simulink model "gtm_design"  (R2021b)
settings: Solver=VariableStepAuto  StartTime=0.0  StopTime=10.0  MinStep=0.00999  RelTol=1e-3
StopFcn:
  | MWSout=grabmws(bdroot);
  | MWSout.lastrun=datestr(now);
values from neighbouring files (symbols this model uses):
  knots2fps = 1.68781    [setup.m]
  s = tf('s')    [setup.m]
undefined symbols (not defined in the file or in its folder): Aero, aftfuel, aftfuel_pos, AILL, AILLC, AILR, AILRC, alpha_deg, alt0, altitude_ft, Ax_g, Ay_g, Az_g, b, beta_deg, bias, BRAKEC, Cbar, cg_pos0, cg_shift_gear, ControlMode, DamageCase, DamageModels, DamageOnsetTime, deltc, Earth, ELLIB, ELLIBC, ELLOB, ELLOBC, ELRIB, ELRIBC, ELROB, ELROBC, engl_ang, engl_pos, engr_ang, engr_pos, etas0, etas1, etasc_feedthrough, FLAPLC, FLAPLIB, FLAPLOB, FLAPRC, FLAPRIB, FLAPROB, FlightMode, FuelUsed_Init, fwdfuel, fwdfuel_pos, GEAR, GEARC, Inertia0, Inertia_shift_gear, Ixx_model, Iyy_model, Izz_model, KTAS, LandingGear ... (+66)
libraries: simulink_extras x98, LPVBlockLibrary x54, simulink_need_slupdate x30, aerolibconvert2 x27, simulink x7, aerolibtransform2 x6, uavalgslib x4, UserContent_lib x2, robotcorelib x1, uavutilslib x1
(part 3 of 9)

== system gtm_design/GTM_T2/Actuators/Acutator Dynamics ==
  In : Inport
  Brake : Saturate  UpperLimit=100  LowerLimit=0
  Bus Selector2 : BusSelector  OutputSignals=ELLOBC,ELLIBC,ELROBC,ELRIBC,AILLC,AILRC,RUDUPC,RUDLOC,SPLLIBC,SPLLOBC,SPLRIBC,SPLROBC,FLAPLC,MORPHLC,FLAPRC,MORPHRC,GEARC,BRAKEC,THROTLC,THROTRC,STEERC
  ElevatorLIBServo : Subsystem  mask(Rate and Position Limited Servo){freq=5, RL=300, POS_hi=20, POS_lo=-30, Bias=bias.elevator}
      mask prompts: freq "Bandwidth, Hz"; RL "Rate Limit:"; POS_hi "Position Limit High:"; POS_lo "Position Limit Low:"; Bias "Bias Value:"
      mask help:
      | First order transfer function: w/(s+w), with rate and position limits
      | and output bias level.
      mask Display:
      | text(.48,.55,sprintf('%3.1f Hz\nBW',freq),'horizontalAlignment','center');
      | 
      | text(0.18,0.45,sprintf('|d/dt|\n<%0.1f',RL),'horizontalAlignment','center');
      | 
      | text(0.88,0.85,num2str(POS_hi),'horizontalAlignment', 'center');
      | text(0.88,0.2,num2str(POS_lo),'horizontalAlignment', 'center');
      | text(0.73,0.5,'P\nL');
      | 
      | 
      | plot([0.83 0.87 0.93 0.97],[0.4 0.4 0.6 0.6]);
      | plot([0.81 0.99],[0.5 0.5]);
      | plot([0.9 0.9],[0.3 0.7]);
      | plot([0.81 0.99 0.99 0.81 0.81],[0.3 0.3 0.7 0.7 0.3]);
  ElevatorLOBServo : Subsystem  mask(Rate and Position Limited Servo){freq=5, RL=300, POS_hi=20, POS_lo=-30, Bias=bias.elevator}
      mask prompts: freq "Bandwidth, Hz"; RL "Rate Limit:"; POS_hi "Position Limit High:"; POS_lo "Position Limit Low:"; Bias "Bias Value:"
      mask help:
      | First order transfer function: w/(s+w), with rate and position limits
      | and output bias level.
      mask Display:
      | text(.48,.55,sprintf('%3.1f Hz\nBW',freq),'horizontalAlignment','center');
      | 
      | text(0.18,0.45,sprintf('|d/dt|\n<%0.1f',RL),'horizontalAlignment','center');
      | 
      | text(0.88,0.85,num2str(POS_hi),'horizontalAlignment', 'center');
      | text(0.88,0.2,num2str(POS_lo),'horizontalAlignment', 'center');
      | text(0.73,0.5,'P\nL');
      | 
      | 
      | plot([0.83 0.87 0.93 0.97],[0.4 0.4 0.6 0.6]);
      | plot([0.81 0.99],[0.5 0.5]);
      | plot([0.9 0.9],[0.3 0.7]);
      | plot([0.81 0.99 0.99 0.81 0.81],[0.3 0.3 0.7 0.7 0.3]);
  ElevatorRIBServo : Subsystem  mask(Rate and Position Limited Servo){freq=5, RL=300, POS_hi=20, POS_lo=-30, Bias=bias.elevator}
      mask prompts: freq "Bandwidth, Hz"; RL "Rate Limit:"; POS_hi "Position Limit High:"; POS_lo "Position Limit Low:"; Bias "Bias Value:"
      mask help:
      | First order transfer function: w/(s+w), with rate and position limits
      | and output bias level.
      mask Display:
      | text(.48,.55,sprintf('%3.1f Hz\nBW',freq),'horizontalAlignment','center');
      | 
      | text(0.18,0.45,sprintf('|d/dt|\n<%0.1f',RL),'horizontalAlignment','center');
      | 
      | text(0.88,0.85,num2str(POS_hi),'horizontalAlignment', 'center');
      | text(0.88,0.2,num2str(POS_lo),'horizontalAlignment', 'center');
      | text(0.73,0.5,'P\nL');
      | 
      | 
      | plot([0.83 0.87 0.93 0.97],[0.4 0.4 0.6 0.6]);
      | plot([0.81 0.99],[0.5 0.5]);
      | plot([0.9 0.9],[0.3 0.7]);
      | plot([0.81 0.99 0.99 0.81 0.81],[0.3 0.3 0.7 0.7 0.3]);
  ElevatorROBServo : Subsystem  mask(Rate and Position Limited Servo){freq=5, RL=300, POS_hi=20, POS_lo=-30, Bias=bias.elevator}
      mask prompts: freq "Bandwidth, Hz"; RL "Rate Limit:"; POS_hi "Position Limit High:"; POS_lo "Position Limit Low:"; Bias "Bias Value:"
      mask help:
      | First order transfer function: w/(s+w), with rate and position limits
      | and output bias level.
      mask Display:
      | text(.48,.55,sprintf('%3.1f Hz\nBW',freq),'horizontalAlignment','center');
      | 
      | text(0.18,0.45,sprintf('|d/dt|\n<%0.1f',RL),'horizontalAlignment','center');
      | 
      | text(0.88,0.85,num2str(POS_hi),'horizontalAlignment', 'center');
      | text(0.88,0.2,num2str(POS_lo),'horizontalAlignment', 'center');
      | text(0.73,0.5,'P\nL');
      | 
      | 
      | plot([0.83 0.87 0.93 0.97],[0.4 0.4 0.6 0.6]);
      | plot([0.81 0.99],[0.5 0.5]);
      | plot([0.9 0.9],[0.3 0.7]);
      | plot([0.81 0.99 0.99 0.81 0.81],[0.3 0.3 0.7 0.7 0.3]);
  FlapLServo : Subsystem  mask(Rate and Position Limited Servo){freq=5, RL=300, POS_hi=30, POS_lo=0, Bias=bias.morphing}
      mask prompts: freq "Bandwidth, Hz"; RL "Rate Limit:"; POS_hi "Position Limit High:"; POS_lo "Position Limit Low:"; Bias "Bias Value:"
      mask help:
      | First order transfer function: w/(s+w), with rate and position limits
      | and output bias level.
      mask Display:
      | text(.48,.55,sprintf('%3.1f Hz\nBW',freq),'horizontalAlignment','center');
      | 
      | text(0.18,0.45,sprintf('|d/dt|\n<%0.1f',RL),'horizontalAlignment','center');
      | 
      | text(0.88,0.85,num2str(POS_hi),'horizontalAlignment', 'center');
      | text(0.88,0.2,num2str(POS_lo),'horizontalAlignment', 'center');
      | text(0.73,0.5,'P\nL');
      | 
      | 
      | plot([0.83 0.87 0.93 0.97],[0.4 0.4 0.6 0.6]);
      | plot([0.81 0.99],[0.5 0.5]);
      | plot([0.9 0.9],[0.3 0.7]);
      | plot([0.81 0.99 0.99 0.81 0.81],[0.3 0.3 0.7 0.7 0.3]);
  FlapRServo : Subsystem  mask(Rate and Position Limited Servo){freq=5, RL=300, POS_hi=30, POS_lo=0, Bias=bias.morphing}
      mask prompts: freq "Bandwidth, Hz"; RL "Rate Limit:"; POS_hi "Position Limit High:"; POS_lo "Position Limit Low:"; Bias "Bias Value:"
      mask help:
      | First order transfer function: w/(s+w), with rate and position limits
      | and output bias level.
      mask Display:
      | text(.48,.55,sprintf('%3.1f Hz\nBW',freq),'horizontalAlignment','center');
      | 
      | text(0.18,0.45,sprintf('|d/dt|\n<%0.1f',RL),'horizontalAlignment','center');
      | 
      | text(0.88,0.85,num2str(POS_hi),'horizontalAlignment', 'center');
      | text(0.88,0.2,num2str(POS_lo),'horizontalAlignment', 'center');
      | text(0.73,0.5,'P\nL');
      | 
      | 
      | plot([0.83 0.87 0.93 0.97],[0.4 0.4 0.6 0.6]);
      | plot([0.81 0.99],[0.5 0.5]);
      | plot([0.9 0.9],[0.3 0.7]);
      | plot([0.81 0.99 0.99 0.81 0.81],[0.3 0.3 0.7 0.7 0.3]);
  Gear : Saturate  UpperLimit=1  LowerLimit=0
  L Throttle : Saturate  UpperLimit=100  LowerLimit=0
  LeftAileronServo : Subsystem  mask(Rate and Position Limited Servo){freq=5, RL=300, POS_hi=20.0, POS_lo=-20, Bias=-1*bias.aileron}
      mask prompts: freq "Bandwidth, Hz"; RL "Rate Limit:"; POS_hi "Position Limit High:"; POS_lo "Position Limit Low:"; Bias "Bias Value:"
      mask help:
      | First order transfer function: w/(s+w), with rate and position limits
      | and output bias level.
      mask Display:
      | text(.48,.55,sprintf('%3.1f Hz\nBW',freq),'horizontalAlignment','center');
      | 
      | text(0.18,0.45,sprintf('|d/dt|\n<%0.1f',RL),'horizontalAlignment','center');
      | 
      | text(0.88,0.85,num2str(POS_hi),'horizontalAlignment', 'center');
      | text(0.88,0.2,num2str(POS_lo),'horizontalAlignment', 'center');
      | text(0.73,0.5,'P\nL');
      | 
      | 
      | plot([0.83 0.87 0.93 0.97],[0.4 0.4 0.6 0.6]);
      | plot([0.81 0.99],[0.5 0.5]);
      | plot([0.9 0.9],[0.3 0.7]);
      | plot([0.81 0.99 0.99 0.81 0.81],[0.3 0.3 0.7 0.7 0.3]);
  LeftIBSpoilerServo : Subsystem  mask(Rate and Position Limited Servo){freq=5, RL=300, POS_hi=15, POS_lo=0, Bias=bias.morphing}
      mask prompts: freq "Bandwidth, Hz"; RL "Rate Limit:"; POS_hi "Position Limit High:"; POS_lo "Position Limit Low:"; Bias "Bias Value:"
      mask help:
      | First order transfer function: w/(s+w), with rate and position limits
      | and output bias level.
      mask Display:
      | text(.48,.55,sprintf('%3.1f Hz\nBW',freq),'horizontalAlignment','center');
      | 
      | text(0.18,0.45,sprintf('|d/dt|\n<%0.1f',RL),'horizontalAlignment','center');
      | 
      | text(0.88,0.85,num2str(POS_hi),'horizontalAlignment', 'center');
      | text(0.88,0.2,num2str(POS_lo),'horizontalAlignment', 'center');
      | text(0.73,0.5,'P\nL');
      | 
      | 
      | plot([0.83 0.87 0.93 0.97],[0.4 0.4 0.6 0.6]);
      | plot([0.81 0.99],[0.5 0.5]);
      | plot([0.9 0.9],[0.3 0.7]);
      | plot([0.81 0.99 0.99 0.81 0.81],[0.3 0.3 0.7 0.7 0.3]);
  LeftOBSpoilerServo : Subsystem  mask(Rate and Position Limited Servo){freq=5, RL=300, POS_hi=45, POS_lo=0, Bias=bias.speedbrake}
      mask prompts: freq "Bandwidth, Hz"; RL "Rate Limit:"; POS_hi "Position Limit High:"; POS_lo "Position Limit Low:"; Bias "Bias Value:"
      mask help:
      | First order transfer function: w/(s+w), with rate and position limits
      | and output bias level.
      mask Display:
      | text(.48,.55,sprintf('%3.1f Hz\nBW',freq),'horizontalAlignment','center');
      | 
      | text(0.18,0.45,sprintf('|d/dt|\n<%0.1f',RL),'horizontalAlignment','center');
      | 
      | text(0.88,0.85,num2str(POS_hi),'horizontalAlignment', 'center');
      | text(0.88,0.2,num2str(POS_lo),'horizontalAlignment', 'center');
      | text(0.73,0.5,'P\nL');
      | 
      | 
      | plot([0.83 0.87 0.93 0.97],[0.4 0.4 0.6 0.6]);
      | plot([0.81 0.99],[0.5 0.5]);
      | plot([0.9 0.9],[0.3 0.7]);
      | plot([0.81 0.99 0.99 0.81 0.81],[0.3 0.3 0.7 0.7 0.3]);
  LeftSpanServo : Subsystem  mask(Rate and Position Limited Servo){freq=5, RL=25, POS_hi=0, POS_lo=-25, Bias=bias.morphing}
      mask prompts: freq "Bandwidth, Hz"; RL "Rate Limit:"; POS_hi "Position Limit High:"; POS_lo "Position Limit Low:"; Bias "Bias Value:"
      mask help:
      | First order transfer function: w/(s+w), with rate and position limits
      | and output bias level.
      mask Display:
      | text(.48,.55,sprintf('%3.1f Hz\nBW',freq),'horizontalAlignment','center');
      | 
      | text(0.18,0.45,sprintf('|d/dt|\n<%0.1f',RL),'horizontalAlignment','center');
      | 
      | text(0.88,0.85,num2str(POS_hi),'horizontalAlignment', 'center');
      | text(0.88,0.2,num2str(POS_lo),'horizontalAlignment', 'center');
      | text(0.73,0.5,'P\nL');
      | 
      | 
      | plot([0.83 0.87 0.93 0.97],[0.4 0.4 0.6 0.6]);
      | plot([0.81 0.99],[0.5 0.5]);
      | plot([0.9 0.9],[0.3 0.7]);
      | plot([0.81 0.99 0.99 0.81 0.81],[0.3 0.3 0.7 0.7 0.3]);
  Mux : Mux  Inputs=21
  R Throttle : Saturate  UpperLimit=100  LowerLimit=0
  RightAileronServo : Subsystem  mask(Rate and Position Limited Servo){freq=5, RL=300, POS_hi=20.0, POS_lo=-20, Bias=bias.aileron}
      mask prompts: freq "Bandwidth, Hz"; RL "Rate Limit:"; POS_hi "Position Limit High:"; POS_lo "Position Limit Low:"; Bias "Bias Value:"
      mask help:
      | First order transfer function: w/(s+w), with rate and position limits
      | and output bias level.
      mask Display:
      | text(.48,.55,sprintf('%3.1f Hz\nBW',freq),'horizontalAlignment','center');
      | 
      | text(0.18,0.45,sprintf('|d/dt|\n<%0.1f',RL),'horizontalAlignment','center');
      | 
      | text(0.88,0.85,num2str(POS_hi),'horizontalAlignment', 'center');
      | text(0.88,0.2,num2str(POS_lo),'horizontalAlignment', 'center');
      | text(0.73,0.5,'P\nL');
      | 
      | 
      | plot([0.83 0.87 0.93 0.97],[0.4 0.4 0.6 0.6]);
      | plot([0.81 0.99],[0.5 0.5]);
      | plot([0.9 0.9],[0.3 0.7]);
      | plot([0.81 0.99 0.99 0.81 0.81],[0.3 0.3 0.7 0.7 0.3]);
  RightIBSpoilerServo : Subsystem  mask(Rate and Position Limited Servo){freq=5, RL=300, POS_hi=15, POS_lo=0, Bias=bias.morphing}
      mask prompts: freq "Bandwidth, Hz"; RL "Rate Limit:"; POS_hi "Position Limit High:"; POS_lo "Position Limit Low:"; Bias "Bias Value:"
      mask help:
      | First order transfer function: w/(s+w), with rate and position limits
      | and output bias level.
      mask Display:
      | text(.48,.55,sprintf('%3.1f Hz\nBW',freq),'horizontalAlignment','center');
      | 
      | text(0.18,0.45,sprintf('|d/dt|\n<%0.1f',RL),'horizontalAlignment','center');
      | 
      | text(0.88,0.85,num2str(POS_hi),'horizontalAlignment', 'center');
      | text(0.88,0.2,num2str(POS_lo),'horizontalAlignment', 'center');
      | text(0.73,0.5,'P\nL');
      | 
      | 
      | plot([0.83 0.87 0.93 0.97],[0.4 0.4 0.6 0.6]);
      | plot([0.81 0.99],[0.5 0.5]);
      | plot([0.9 0.9],[0.3 0.7]);
      | plot([0.81 0.99 0.99 0.81 0.81],[0.3 0.3 0.7 0.7 0.3]);
  RightOBSpoilerServo : Subsystem  mask(Rate and Position Limited Servo){freq=5, RL=300, POS_hi=45, POS_lo=0, Bias=bias.speedbrake}
      mask prompts: freq "Bandwidth, Hz"; RL "Rate Limit:"; POS_hi "Position Limit High:"; POS_lo "Position Limit Low:"; Bias "Bias Value:"
      mask help:
      | First order transfer function: w/(s+w), with rate and position limits
      | and output bias level.
      mask Display:
      | text(.48,.55,sprintf('%3.1f Hz\nBW',freq),'horizontalAlignment','center');
      | 
      | text(0.18,0.45,sprintf('|d/dt|\n<%0.1f',RL),'horizontalAlignment','center');
      | 
      | text(0.88,0.85,num2str(POS_hi),'horizontalAlignment', 'center');
      | text(0.88,0.2,num2str(POS_lo),'horizontalAlignment', 'center');
      | text(0.73,0.5,'P\nL');
      | 
      | 
      | plot([0.83 0.87 0.93 0.97],[0.4 0.4 0.6 0.6]);
      | plot([0.81 0.99],[0.5 0.5]);
      | plot([0.9 0.9],[0.3 0.7]);
      | plot([0.81 0.99 0.99 0.81 0.81],[0.3 0.3 0.7 0.7 0.3]);
  RightSpanServo : Subsystem  mask(Rate and Position Limited Servo){freq=5, RL=25, POS_hi=0, POS_lo=-25, Bias=bias.morphing}
      mask prompts: freq "Bandwidth, Hz"; RL "Rate Limit:"; POS_hi "Position Limit High:"; POS_lo "Position Limit Low:"; Bias "Bias Value:"
      mask help:
      | First order transfer function: w/(s+w), with rate and position limits
      | and output bias level.
      mask Display:
      | text(.48,.55,sprintf('%3.1f Hz\nBW',freq),'horizontalAlignment','center');
      | 
      | text(0.18,0.45,sprintf('|d/dt|\n<%0.1f',RL),'horizontalAlignment','center');
      | 
      | text(0.88,0.85,num2str(POS_hi),'horizontalAlignment', 'center');
      | text(0.88,0.2,num2str(POS_lo),'horizontalAlignment', 'center');
      | text(0.73,0.5,'P\nL');
      | 
      | 
      | plot([0.83 0.87 0.93 0.97],[0.4 0.4 0.6 0.6]);
      | plot([0.81 0.99],[0.5 0.5]);
      | plot([0.9 0.9],[0.3 0.7]);
      | plot([0.81 0.99 0.99 0.81 0.81],[0.3 0.3 0.7 0.7 0.3]);
  RudderLServo : Subsystem  mask(Rate and Position Limited Servo){freq=5, RL=300, POS_hi=30, POS_lo=-30.0, Bias=bias.rudder}
      mask prompts: freq "Bandwidth, Hz"; RL "Rate Limit:"; POS_hi "Position Limit High:"; POS_lo "Position Limit Low:"; Bias "Bias Value:"
      mask help:
      | First order transfer function: w/(s+w), with rate and position limits
      | and output bias level.
      mask Display:
      | text(.48,.55,sprintf('%3.1f Hz\nBW',freq),'horizontalAlignment','center');
      | 
      | text(0.18,0.45,sprintf('|d/dt|\n<%0.1f',RL),'horizontalAlignment','center');
      | 
      | text(0.88,0.85,num2str(POS_hi),'horizontalAlignment', 'center');
      | text(0.88,0.2,num2str(POS_lo),'horizontalAlignment', 'center');
      | text(0.73,0.5,'P\nL');
      | 
      | 
      | plot([0.83 0.87 0.93 0.97],[0.4 0.4 0.6 0.6]);
      | plot([0.81 0.99],[0.5 0.5]);
      | plot([0.9 0.9],[0.3 0.7]);
      | plot([0.81 0.99 0.99 0.81 0.81],[0.3 0.3 0.7 0.7 0.3]);
  RudderUServo : Subsystem  mask(Rate and Position Limited Servo){freq=5, RL=300, POS_hi=30, POS_lo=-30.0, Bias=bias.rudder}
      mask prompts: freq "Bandwidth, Hz"; RL "Rate Limit:"; POS_hi "Position Limit High:"; POS_lo "Position Limit Low:"; Bias "Bias Value:"
      mask help:
      | First order transfer function: w/(s+w), with rate and position limits
      | and output bias level.
      mask Display:
      | text(.48,.55,sprintf('%3.1f Hz\nBW',freq),'horizontalAlignment','center');
      | 
      | text(0.18,0.45,sprintf('|d/dt|\n<%0.1f',RL),'horizontalAlignment','center');
      | 
      | text(0.88,0.85,num2str(POS_hi),'horizontalAlignment', 'center');
      | text(0.88,0.2,num2str(POS_lo),'horizontalAlignment', 'center');
      | text(0.73,0.5,'P\nL');
      | 
      | 
      | plot([0.83 0.87 0.93 0.97],[0.4 0.4 0.6 0.6]);
      | plot([0.81 0.99],[0.5 0.5]);
      | plot([0.9 0.9],[0.3 0.7]);
      | plot([0.81 0.99 0.99 0.81 0.81],[0.3 0.3 0.7 0.7 0.3]);
  SteeringServo : Subsystem  mask(Rate and Position Limited Servo){freq=10, RL=300, POS_hi=30, POS_lo=-30, Bias=0}
      mask prompts: freq "Bandwidth, Hz"; RL "Rate Limit:"; POS_hi "Position Limit High:"; POS_lo "Position Limit Low:"; Bias "Bias Value:"
      mask help:
      | First order transfer function: w/(s+w), with rate and position limits
      | and output bias level.
      mask Display:
      | text(.48,.55,sprintf('%3.1f Hz\nBW',freq),'horizontalAlignment','center');
      | 
      | text(0.18,0.45,sprintf('|d/dt|\n<%0.1f',RL),'horizontalAlignment','center');
      | 
      | text(0.88,0.85,num2str(POS_hi),'horizontalAlignment', 'center');
      | text(0.88,0.2,num2str(POS_lo),'horizontalAlignment', 'center');
      | text(0.73,0.5,'P\nL');
      | 
      | 
      | plot([0.83 0.87 0.93 0.97],[0.4 0.4 0.6 0.6]);
      | plot([0.81 0.99],[0.5 0.5]);
      | plot([0.9 0.9],[0.3 0.7]);
      | plot([0.81 0.99 0.99 0.81 0.81],[0.3 0.3 0.7 0.7 0.3]);
  Sum : Sum  Inputs=++|
  Sum1 : Sum  Inputs=++|
  Sum2 : Sum  Inputs=++|
  Throttle : Constant  Value=bias.throttle
  Throttle1 : Constant  Value=bias.throttle
  Throttle2 : Constant  Value=bias.geardown
  Out : Outport
  wires:
  Bus Selector2/17 -> Sum2/2  "<GEARC>"
  Throttle2/1 -> Sum2/1
  Sum2/1 -> Gear/1
  Bus Selector2/20 -> Sum1/2  "<THROTRC>"
  Throttle1/1 -> Sum1/1
  Sum1/1 -> R Throttle/1
  Bus Selector2/19 -> Sum/2  "<THROTLC>"
  Throttle/1 -> Sum/1
  Sum/1 -> L Throttle/1
  SteeringServo/1(Out) -> Mux/21
  R Throttle/1 -> Mux/20
  L Throttle/1 -> Mux/19
  Brake/1 -> Mux/18
  Gear/1 -> Mux/17
  Mux/1 -> Out/1
  In/1 -> Bus Selector2/1
  Bus Selector2/21 -> SteeringServo/1(In)  "<STEERC>"
  RightSpanServo/1(Out) -> Mux/16
  FlapRServo/1(Out) -> Mux/15
  FlapLServo/1(Out) -> Mux/13
  RightOBSpoilerServo/1(Out) -> Mux/12
  RightIBSpoilerServo/1(Out) -> Mux/11
  LeftIBSpoilerServo/1(Out) -> Mux/9
  RudderLServo/1(Out) -> Mux/8
  Bus Selector2/12 -> RightOBSpoilerServo/1(In)  "<SPLROBC>"
  Bus Selector2/11 -> RightIBSpoilerServo/1(In)  "<SPLRIBC>"
  Bus Selector2/9 -> LeftIBSpoilerServo/1(In)  "<SPLLIBC>"
  Bus Selector2/8 -> RudderLServo/1(In)  "<RUDLOC>"
  Bus Selector2/7 -> RudderUServo/1(In)  "<RUDUPC>"
  RudderUServo/1(Out) -> Mux/7  "RUD"
  RightAileronServo/1(Out) -> Mux/6  "AILR"
  Bus Selector2/6 -> RightAileronServo/1(In)  "<AILRC>"
  LeftAileronServo/1(Out) -> Mux/5  "AILL"
  Bus Selector2/5 -> LeftAileronServo/1(In)  "<AILLC>"
  ElevatorRIBServo/1(Out) -> Mux/4
  Bus Selector2/4 -> ElevatorRIBServo/1(In)  "<ELRIBC>"
  ElevatorROBServo/1(Out) -> Mux/3
  Bus Selector2/3 -> ElevatorROBServo/1(In)  "<ELROBC>"
  ElevatorLIBServo/1(Out) -> Mux/2
  ElevatorLOBServo/1(Out) -> Mux/1  "ELL"
  Bus Selector2/2 -> ElevatorLIBServo/1(In)  "<ELLIBC>"
  Bus Selector2/1 -> ElevatorLOBServo/1(In)  "<ELLOBC>"
  Bus Selector2/18 -> Brake/1  "<BRAKEC>"
  Bus Selector2/16 -> RightSpanServo/1(In)  "<MORPHRC>"
  Bus Selector2/15 -> FlapRServo/1(In)  "<FLAPRC>"
  Bus Selector2/14 -> LeftSpanServo/1(In)  "<MORPHLC>"
  Bus Selector2/13 -> FlapLServo/1(In)  "<FLAPLC>"
  Bus Selector2/10 -> LeftOBSpoilerServo/1(In)  "<SPLLOBC>"
  LeftOBSpoilerServo/1(Out) -> Mux/10
  LeftSpanServo/1(Out) -> Mux/14

== system gtm_design/GTM_T2/Actuators/DeadBand ==
  I : Inport
  Deadband : Subsystem
  Flaps : Constant  Value=SurfaceDeadbandOn
  Switch : Switch  Criteria=u2 ~= 0  Threshold=0.2
  O : Outport
  wires:
  I/1 -> Switch/3, Deadband/1(In)
  Deadband/1(Out) -> Switch/1
  Switch/1 -> O/1
  Flaps/1 -> Switch/2

== system gtm_design/GTM_T2/Actuators/InputModification for Trimming ==
  CmdVec : Inport
  SurfBias : Inport  Port=2
  SurfaceDeltas : Inport  Port=3
  Clock : Clock
  Compare To Constant : simulink/Logic and Bit Operations/Compare To Constant  relop=>=  const=0.2  OutDataTypeStr=boolean  ZeroCross=off
  Constant : Constant  Value=TrimModeOn
  Constant1 : Constant  Value=LinearizeModeOn
  Constant2 : Constant  Value=TrimModeOn
  Constant3 : Constant  Value=LinearizeModeOn
  Gain : Gain  Gain=2
  "Invalid, Error Out" : Subsystem  TreatAsAtomicUnit=on
  KillifNotSimMode : Assertion  AssertionFailFcn="warndlg('Running simulation with TrimMode or LinearizeMode engaged.  Run setup.m to reset.','Warning!')"
  LinearizeMode:DetlasOnTrimBias : Subsystem  TreatAsAtomicUnit=on
  Logical Operator : Logic  Operator=NAND  AllPortsSameDT=off  OutDataTypeStr=boolean
  Logical Operator1 : Logic  Operator=OR  AllPortsSameDT=off  OutDataTypeStr=boolean
  Merge : Merge  Inputs=4  InitialOutput=zeros(22,1)
  SimMode:PassThroughWithStab : Subsystem  TreatAsAtomicUnit=on
  Sum : Sum  Inputs=|++
  Switch Case : SwitchCase  CaseConditions={0,1,2}
  TrimMode: DriveFromTopLevel : Subsystem  TreatAsAtomicUnit=on
  CmdVecOut : Outport
  wires:
  "Invalid, Error Out"/1(Out) -> Merge/4
  Compare To Constant/1 -> Logical Operator/2
  Logical Operator1/1 -> Logical Operator/1
  Constant2/1 -> Logical Operator1/1
  Constant3/1 -> Logical Operator1/2
  Logical Operator/1 -> KillifNotSimMode/1
  Clock/1 -> Compare To Constant/1
  Switch Case/4 -> "Invalid, Error Out"/Action
  Sum/1 -> Switch Case/1
  Gain/1 -> Sum/2
  Constant/1 -> Sum/1
  Constant1/1 -> Gain/1
  LinearizeMode:DetlasOnTrimBias/1(Out) -> Merge/3
  SurfaceDeltas/1 -> LinearizeMode:DetlasOnTrimBias/1(In1)
  Switch Case/3 -> LinearizeMode:DetlasOnTrimBias/Action
  Merge/1 -> CmdVecOut/1
  TrimMode: DriveFromTopLevel/1(Out) -> Merge/2
  SimMode:PassThroughWithStab/1(Out) -> Merge/1
  SurfBias/1 -> TrimMode: DriveFromTopLevel/1(TrimBias)
  Switch Case/2 -> TrimMode: DriveFromTopLevel/Action
  Switch Case/1 -> SimMode:PassThroughWithStab/Action
  CmdVec/1 -> SimMode:PassThroughWithStab/1(Cmd)

== system gtm_design/GTM_T2/Actuators/Label ==
  I : Inport
  Bus Creator : BusCreator  Inputs=22
  Demux : Demux  Outputs=22
  O : Outport
  wires:
  Demux/22 -> Bus Creator/22  "STEER"
  Demux/21 -> Bus Creator/21  "THROTR"
  Demux/20 -> Bus Creator/20  "THROTL"
  Demux/19 -> Bus Creator/19  "BRAKE"
  Demux/1 -> Bus Creator/1  "ELLOB"
  Demux/18 -> Bus Creator/18  "GEAR"
  Demux/17 -> Bus Creator/17  "STAB"
  Demux/16 -> Bus Creator/16  "FLAPROB"
  Demux/15 -> Bus Creator/15  "FLAPRIB"
  Demux/14 -> Bus Creator/14  "FLAPLOB"
  Demux/13 -> Bus Creator/13  "FLAPLIB"
  Demux/12 -> Bus Creator/12  "SPLROB"
  Demux/11 -> Bus Creator/11  "SPLRIB"
  Demux/10 -> Bus Creator/10  "SPLLOB"
  Demux/9 -> Bus Creator/9  "SPLLIB"
  Demux/8 -> Bus Creator/8  "RUDL"
  Demux/7 -> Bus Creator/7  "RUDU"
  Demux/6 -> Bus Creator/6  "AILR"
  Demux/5 -> Bus Creator/5  "AILL"
  Demux/4 -> Bus Creator/4  "ELRIB"
  Demux/3 -> Bus Creator/3  "ELROB"
  Demux/2 -> Bus Creator/2  "ELLIB"
  Bus Creator/1 -> O/1
  I/1 -> Demux/1

== system gtm_design/GTM_T2/Actuators/TimeDelay with IC feedthrough ==
  I : Inport
  Clock : Clock
  Demux : Demux  Outputs=[16 5]
  Mux : Mux  Inputs=[16 5]
  Switch : Switch  Threshold=10.1e-3
  Transport Delay : TransportDelay  DelayTime=10e-3
      settings: AttributesFormatString=%<DelayTime>
  O : Outport
  wires:
  Mux/1 -> Switch/1
  Demux/2 -> Mux/2
  Transport Delay/1 -> Mux/1
  Demux/1 -> Transport Delay/1
  Switch/1 -> O/1
  Clock/1 -> Switch/2
  I/1 -> Demux/1, Switch/3

== system gtm_design/GTM_T2/Aero/Basic Airframe ==
  note: The basic aerodynamics are asymmetric.
      | When the 'symmetry_on' flag is set, increments
      | from the dC3_sym aero table are added to the
      | lateral-directional coefficients (CY,Cl,Cn) to make
      | them symmetric.  When the flag is off, the gain of
      | 2.0 is applied to the increments,which effectively
      | changes the sign of the asymmetries.
  alpha : Inport
  beta : Inport  Port=2
  symmetry_on : Inport  Port=3
  AC_Params : Inport  Port=4
  Add : Sum  Inputs=+++
  AlphaLookup : PreLookup  BreakpointsData=Aero.C6_bas.alpha  IndexSearchMethod=Linear search  BeginIndexSearchUsingPreviousIndexResult=on  ExtrapMethod=Linear
  AlphaLookup1 : PreLookup  BreakpointsData=Aero.C6_bas.beta  IndexSearchMethod=Linear search  BeginIndexSearchUsingPreviousIndexResult=on  ExtrapMethod=Linear
  Assignment to Lateral : Assignment  IndexMode=Zero-based  IndexOptions=Index vector (dialog)  Indices=[1 3 5]  OutputSizes=[1 1]
  Bus Selector : BusSelector  OutputSignals=DamageCase
  Constant : Constant  Value=zeros(6,1)
  Constant1 : Constant  Value=[0:5]  OutDataTypeStr=uint32
  Constant2 : Constant  Value=[0:2]  OutDataTypeStr=uint32
  DamageEffects : Subsystem
  Data Type Conversion : DataTypeConversion  OutDataTypeStr=uint32  RndMeth=Nearest
  Gain : Gain  Gain=2
  Interpolation Using Prelookup : Interpolation_n-D  NumberOfTableDimensions=3  Table=Aero.C6_bas.data  NumSelectionDims=1
      settings: InputPortMap=u0,u1,u2,u3,u4
  Interpolation Using Prelookup1 : Interpolation_n-D  NumberOfTableDimensions=3  Table=Aero.dC3_sym.data  NumSelectionDims=1
      settings: InputPortMap=u0,u1,u2,u3,u4
  Switch : Switch  Criteria=u2 ~= 0
  C6 : Outport
  wires:
  Assignment to Lateral/1 -> Gain/1, Switch/1
  Data Type Conversion/1 -> DamageEffects/3(damage_case)
  Constant2/1 -> Interpolation Using Prelookup1/5
  Constant1/1 -> Interpolation Using Prelookup/5
  AlphaLookup1/2 -> Interpolation Using Prelookup1/4, Interpolation Using Prelookup/4
  AlphaLookup1/1 -> Interpolation Using Prelookup1/3, Interpolation Using Prelookup/3
  AlphaLookup/2 -> Interpolation Using Prelookup1/2, Interpolation Using Prelookup/2
  AlphaLookup/1 -> Interpolation Using Prelookup1/1, Interpolation Using Prelookup/1
  Bus Selector/1 -> Data Type Conversion/1  "<DamageCase>"
  AC_Params/1 -> Bus Selector/1
  DamageEffects/1(dC6_dam) -> Add/3
  beta/1 -> AlphaLookup1/1, DamageEffects/2(beta)
  alpha/1 -> AlphaLookup/1, DamageEffects/1(alpha)
  Switch/1 -> Add/2
  Add/1 -> C6/1
  symmetry_on/1 -> Switch/2
  Gain/1 -> Switch/3
  Interpolation Using Prelookup1/1 -> Assignment to Lateral/2
  Constant/1 -> Assignment to Lateral/1
  Interpolation Using Prelookup/1 -> Add/1

== system gtm_design/GTM_T2/Aero/Coefficent Evaluation ==
  C6 Body : Inport
  qbar : Inport  Port=2
  Cg : Inport  Port=3
  Cp : Inport  Port=4
  3D Vector Cross Product : Subsystem
  Demux : Demux  Outputs=[3 3]
      settings: DisplayOption=none
  Gain2 : Gain  Gain=Sref  SaturateOnIntegerOverflow=on  OutDataTypeStr=Inherit: Same as input  ParamDataTypeStr=Inherit: Same as input
  Product : Product  InputSameDT=on  SaturateOnIntegerOverflow=on  OutDataTypeStr=Inherit: Same as first input
  Reference Lengths : Gain  Gain=[b cbar b]  SaturateOnIntegerOverflow=on  OutDataTypeStr=Inherit: Same as input  ParamDataTypeStr=Inherit: Same as input
  Sum : Sum  Inputs=-+  SaturateOnIntegerOverflow=on
  Sum1 : Sum  Inputs=++|  SaturateOnIntegerOverflow=on
  Forces : Outport
  Moments : Outport  Port=2
  wires:
  3D Vector Cross Product/1(AxB) -> Sum1/1
  Sum1/1 -> Moments/1
  Reference Lengths/1 -> Sum1/2
  Demux/1 -> Forces/1, 3D Vector Cross Product/2(B)
  Demux/2 -> Reference Lengths/1
  Gain2/1 -> Demux/1
  Product/1 -> Gain2/1
  qbar/1 -> Product/2
  C6 Body/1 -> Product/1
  Cp/1 -> Sum/2
  Cg/1 -> Sum/1
  Sum/1 -> 3D Vector Cross Product/1(A)

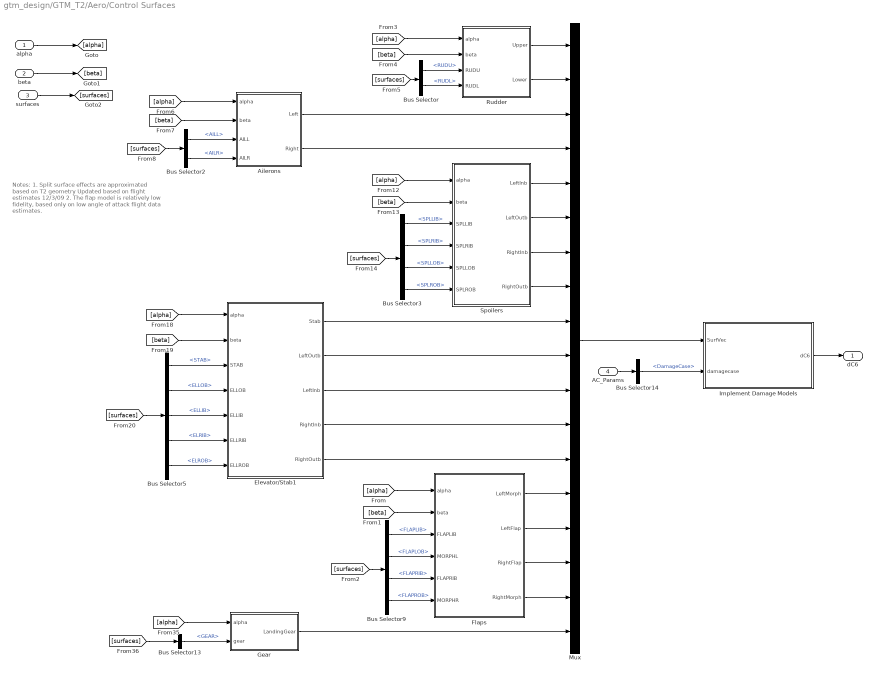
== system gtm_design/GTM_T2/Aero/Control Surfaces ==
  note: Notes:
      | 1. Split surface effects are approximated
      | based on T2 geometry
      | Updated based on flight estimates 12/3/09
      |
      | 2. The flap model is relatively low fidelity, based
      | only on low angle of attack flight data estimates.
  alpha : Inport
  beta : Inport  Port=2  PortDimensions=1
  surfaces : Inport  Port=3
  AC_Params : Inport  Port=4
  Ailerons : Subsystem
  Bus Selector : BusSelector  OutputSignals=RUDU,RUDL
  Bus Selector13 : BusSelector  OutputSignals=GEAR
  Bus Selector14 : BusSelector  OutputSignals=DamageCase
  Bus Selector2 : BusSelector  OutputSignals=AILL,AILR
  Bus Selector3 : BusSelector  OutputSignals=SPLLIB,SPLRIB,SPLLOB,SPLROB
  Bus Selector5 : BusSelector  OutputSignals=STAB,ELLOB,ELLIB,ELRIB,ELROB
  Bus Selector9 : BusSelector  OutputSignals=FLAPLIB,FLAPLOB,FLAPRIB,FLAPROB
  Elevator/Stab1 : Subsystem
  Flaps : Subsystem
  Gear : Subsystem
  Implement Damage Models : Subsystem  mask{DamageModels=DamageModels}
      mask prompts: DamageModels "Cell Array of Damage Models"
      mask help: Implements Damage Models as gain and bias effects on selected surfaces.
      mask init:
      | SurfList={...
      |     'RUDU','RUDL',...
      |     'AILL','AILR',...
      |     'SPLLIB','SPLRIB','SPLLOB','SPLROB',...
      |     'STAB',...
      |     'ELLOB','ELLIB','ELRIB','ELROB',...
      |     'FLAPLOB','FALPLIB','FLAPRIB','FLAPROB',...
      |     'GEAR'
      |     };
      | 
      | Ncases=length(DamageModels);
      | Nsurfs=length(SurfList);
      | SurfGain=ones(Ncases,Nsurfs,6);   %Nominally unity gain, zero bias
      | 
      | %If damage case includes gain/bias on a surface adjust nominal values
      | % First damage case is "no damage".
      | for i=1:Ncases,
      |  for j=1:Nsurfs,
      |     if isfield(DamageModels{i},SurfList{j}),
      |         SurfGain(i,j,:)=DamageModels{i}.(SurfList{j}).gain*ones(1,6);
      |     end
      |  end
      | end
  Mux : Mux  Inputs=18
  Rudder : Subsystem
  Spoilers : Subsystem
  dC6 : Outport
  wires:
  Bus Selector9/4 -> Flaps/6(MORPHR)  "<FLAPROB>"
  Bus Selector9/3 -> Flaps/5(FLAPRIB)  "<FLAPRIB>"
  Bus Selector9/1 -> Flaps/3(FLAPLIB)  "<FLAPLIB>"
  Bus Selector9/2 -> Flaps/4(MORPHL)  "<FLAPLOB>"
  Implement Damage Models/1(dC6) -> dC6/1
  Mux/1 -> Implement Damage Models/1(SurfVec)
  Bus Selector14/1 -> Implement Damage Models/2(damagecase)  "<DamageCase>"
  Flaps/4(RightMorph) -> Mux/17
  Flaps/3(RightFlap) -> Mux/16
  Flaps/2(LeftFlap) -> Mux/15
  Flaps/1(LeftMorph) -> Mux/14
  Gear/1(LandingGear) -> Mux/18
  Elevator/Stab1/5(RightOutb) -> Mux/13
  Elevator/Stab1/4(RightInb) -> Mux/12
  Elevator/Stab1/3(LeftInb) -> Mux/11
  Elevator/Stab1/2(LeftOutb) -> Mux/10
  Elevator/Stab1/1(Stab) -> Mux/9
  Spoilers/4(RightOutb) -> Mux/8
  Spoilers/3(RightInb) -> Mux/7
  Spoilers/2(LeftOutb) -> Mux/6
  Spoilers/1(LeftInb) -> Mux/5
  Ailerons/2(Right) -> Mux/4
  Ailerons/1(Left) -> Mux/3
  Rudder/2(Lower) -> Mux/2
  Rudder/1(Upper) -> Mux/1
  Bus Selector5/5 -> Elevator/Stab1/7(ELLROB)  "<ELROB>"
  Bus Selector5/4 -> Elevator/Stab1/6(ELLRIB)  "<ELRIB>"
  Bus Selector5/3 -> Elevator/Stab1/5(ELLIB)  "<ELLIB>"
  Bus Selector3/4 -> Spoilers/6(SPLROB)  "<SPLROB>"
  Bus Selector3/3 -> Spoilers/5(SPLLOB)  "<SPLLOB>"
  AC_Params/1 -> Bus Selector14/1
  alpha/1 -> [alpha]
  beta/1 -> [beta]
  surfaces/1 -> [surfaces]
  [alpha] -> Rudder/1(alpha)
  [beta] -> Rudder/2(beta)
  [surfaces] -> Bus Selector/1
  Bus Selector/1 -> Rudder/3(RUDU)  "<RUDU>"
  Bus Selector/2 -> Rudder/4(RUDL)  "<RUDL>"
  [alpha] -> Ailerons/1(alpha)
  [beta] -> Ailerons/2(beta)
  [surfaces] -> Bus Selector2/1
  Bus Selector2/1 -> Ailerons/3(AILL)  "<AILL>"
  Bus Selector2/2 -> Ailerons/4(AILR)  "<AILR>"
  [alpha] -> Spoilers/1(alpha)
  [beta] -> Spoilers/2(beta)
  [surfaces] -> Bus Selector3/1
  Bus Selector3/1 -> Spoilers/3(SPLLIB)  "<SPLLIB>"
  Bus Selector3/2 -> Spoilers/4(SPLRIB)  "<SPLRIB>"
  [beta] -> Elevator/Stab1/2(beta)
  [surfaces] -> Bus Selector5/1
  [alpha] -> Elevator/Stab1/1(alpha)
  Bus Selector5/1 -> Elevator/Stab1/3(STAB)  "<STAB>"
  Bus Selector5/2 -> Elevator/Stab1/4(ELLOB)  "<ELLOB>"
  [surfaces] -> Bus Selector9/1
  [alpha] -> Flaps/1(alpha)
  [surfaces] -> Bus Selector13/1
  [alpha] -> Gear/1(alpha)
  Bus Selector13/1 -> Gear/2(gear)  "<GEAR>"
  [beta] -> Flaps/2(beta)

== system gtm_design/GTM_T2/Aero/Dynamic Derviatives ==
  alpha : Inport
  beta : Inport  Port=2
  TAS : Inport  Port=3
  pqr : Inport  Port=4
  AC_Params : Inport  Port=5
  AC_Params1 : InportShadow  Port=5
  AC_Params_Dup1 : InportShadow  Port=5
  Bus Selector : BusSelector  OutputSignals=DamageCase
  Data Type Conversion : DataTypeConversion  OutDataTypeStr=uint32  RndMeth=Nearest
  Forced Oscillation with Damage Increments : Subsystem
  Merge : Merge  InitialOutput=zeros(6,1)
  Rotary Blended UnDamaged Case : Subsystem
  Switch Case : SwitchCase  CaseConditions={[1,2,3,4,5,6]}
  TAS1 : InportShadow  Port=3
  alpha_Dup1 : InportShadow
  pqr_Dup1 : InportShadow  Port=4
  dC6 : Outport
  wires:
  Forced Oscillation with Damage Increments/1(dC6) -> Merge/1
  [ndx] -> Forced Oscillation with Damage Increments/5(DamageCase)
  AC_Params1/1 -> Forced Oscillation with Damage Increments/4(AC_Params)
  pqr_Dup1/1 -> Forced Oscillation with Damage Increments/3(pqr)
  TAS1/1 -> Forced Oscillation with Damage Increments/2(TAS)
  alpha_Dup1/1 -> Forced Oscillation with Damage Increments/1(alpha)
  [ndx] -> Switch Case/1
  Data Type Conversion/1 -> [ndx]
  AC_Params_Dup1/1 -> Bus Selector/1
  Bus Selector/1 -> Data Type Conversion/1  "<DamageCase>"
  Rotary Blended UnDamaged Case/1(dC6) -> Merge/2
  Switch Case/2 -> Rotary Blended UnDamaged Case/Action
  Switch Case/1 -> Forced Oscillation with Damage Increments/Action
  Merge/1 -> dC6/1
  AC_Params/1 -> Rotary Blended UnDamaged Case/5(AC_Params)
  pqr/1 -> Rotary Blended UnDamaged Case/4(pqr)
  TAS/1 -> Rotary Blended UnDamaged Case/3(TAS)
  beta/1 -> Rotary Blended UnDamaged Case/2(beta)
  alpha/1 -> Rotary Blended UnDamaged Case/1(alpha)

== system gtm_design/GTM_T2/Aero/Label ==
  If : Inport
  Im : Inport  Port=2
  Bus Creator1 : BusCreator  Inputs=6
  Demux1 : Demux  Outputs=3
      settings: DisplayOption=none
  Demux3 : Demux  Outputs=3
      settings: DisplayOption=none
  O : Outport
  wires:
  Bus Creator1/1 -> O/1
  If/1 -> Demux1/1
  Demux1/1 -> Bus Creator1/1  "XB"
  Demux1/2 -> Bus Creator1/2  "YB"
  Demux1/3 -> Bus Creator1/3  "ZB"
  Demux3/1 -> Bus Creator1/4  "LB"
  Demux3/2 -> Bus Creator1/5  "MB"
  Demux3/3 -> Bus Creator1/6  "NB"
  Im/1 -> Demux3/1

== system gtm_design/GTM_T2/Aero/Stall Rolling Moment Asymmetry ==
  alpha : Inport
  beta : Inport  Port=2
  stall_cl_asym_enabled : Inport  Port=3
  AlphaWindow : Lookup  InputValues="[12.5   13.5   14.5]"  Table="[0  1  0]"  LookUpMeth=Interpolation-Use End Values
  Assignment to Cl : Assignment  IndexMode=Zero-based  IndexOptions=Index vector (dialog)  Indices=3  OutputSizes=[1 1]
  BetaWindow : Lookup  InputValues=[-2 -1 1 2]  Table=[0 1 1 0]  LookUpMeth=Interpolation-Use End Values
  Constant : Constant  Value=zeros(6,1)
  Product1 : Product  RndMeth=Zero
  Switch2 : Switch  Criteria=u2 > Threshold
  stall_cl_asym_coeff : Gain  Gain=0.01
  zero if disabled : Constant  Value=0
  dC6 : Outport
  wires:
  Switch2/1 -> Assignment to Cl/2
  zero if disabled/1 -> Switch2/3
  stall_cl_asym_enabled/1 -> Switch2/2
  Constant/1 -> Assignment to Cl/1
  Assignment to Cl/1 -> dC6/1
  beta/1 -> BetaWindow/1
  AlphaWindow/1 -> Product1/2
  BetaWindow/1 -> Product1/1
  Product1/1 -> stall_cl_asym_coeff/1
  alpha/1 -> AlphaWindow/1
  stall_cl_asym_coeff/1 -> Switch2/1

== system gtm_design/GTM_T2/AuxiliaryVariables/Atmos76 ==
  States : Inport
  Atmos List : Subsystem
  Bus Selector11 : BusSelector  OutputSignals=altitude
  Ground : Ground
  atmos76 : MATLAB Function  TreatAsAtomicUnit=on
  Atmos : Outport
  wires:
  Ground/1 -> atmos76/2(dt)
  Atmos List/1(O) -> Atmos/1
  States/1 -> Bus Selector11/1
  Bus Selector11/1 -> atmos76/1(z)  "<altitude>"
  atmos76/1(y) -> Atmos List/1(I)

== system gtm_design/GTM_T2/AuxiliaryVariables/Euler to DCM ==
  "Euler " : Inport
  Fcn : Fcn  Expr=u(4)*u(2)*u(6)+u(3)*u(1)
  Fcn1 : Fcn  Expr=u(3)*u(5)
  Fcn2 : Fcn  Expr=u(3)*u(2)*u(1)+u(6)*u(4)
  Fcn3 : Fcn  Expr=u(3)*u(2)*u(4)-u(6)*u(1)
  Fcn4 : Fcn  Expr=-u(2)
  Fcn5 : Fcn  Expr=u(5)*u(1)
  Fcn6 : Fcn  Expr=u(1)*u(2)*u(6)-u(3)*u(4)
  Fcn7 : Fcn  Expr=u(5)*u(6)
  Fcn8 : Fcn  Expr=u(5)*u(4)
  Mux : Mux  Inputs=2
  Mux1 : Mux  Inputs=9
  Reshape : Reshape  OutputDimensionality=Customize  OutputDimensions=[3,3]
  Trigonometric Function : Trigonometry
  Trigonometric Function1 : Trigonometry  Operator=cos
  DCM : Outport
  wires:
  "Euler "/1 -> Trigonometric Function1/1, Trigonometric Function/1
  Trigonometric Function/1 -> Mux/1
  Trigonometric Function1/1 -> Mux/2
  Mux/1 -> Fcn4/1, Fcn8/1, Fcn5/1, Fcn3/1, Fcn/1, Fcn7/1, Fcn6/1, Fcn1/1, Fcn2/1
  Mux1/1 -> Reshape/1
  Fcn7/1 -> Mux1/1
  Fcn6/1 -> Mux1/2
  Fcn/1 -> Mux1/3
  Fcn1/1 -> Mux1/4
  Fcn2/1 -> Mux1/5
  Fcn3/1 -> Mux1/6
  Fcn4/1 -> Mux1/7
  Fcn5/1 -> Mux1/8
  Fcn8/1 -> Mux1/9
  Reshape/1 -> DCM/1

== system gtm_design/GTM_T2/AuxiliaryVariables/Map 0_360 ==
  I : Inport
  Constant : Constant  Value=2*pi
  Constant1 : Constant  Value=0
  Gain : Gain  Gain=180/pi
  Sum : Sum  Inputs=|++
  ifnegadd2pi : Switch
  O : Outport
  wires:
  Gain/1 -> O/1
  Constant1/1 -> ifnegadd2pi/1
  Constant/1 -> ifnegadd2pi/3
  ifnegadd2pi/1 -> Sum/2
  Sum/1 -> Gain/1
  I/1 -> ifnegadd2pi/2, Sum/1

== system gtm_design/GTM_T2/AuxiliaryVariables/Vb Converter ==
  Vb : Inport
  Wind_b : Inport  Port=2
  Add : Sum  Inputs=+-
  Demux : Demux  Outputs=3
      settings: DisplayOption=none
  Dot Product : DotProduct  InputSameDT=on  OutDataTypeStr=Inherit: Inherit via internal rule
  Math Function : Math  Operator=sqrt  SignedPower=on  SaturateOnIntegerOverflow=on
  Product : Product  Inputs=/*  SaturateOnIntegerOverflow=on  OutDataTypeStr=Inherit: Same as first input
  Rad to Deg : Gain  Gain=180/pi  SaturateOnIntegerOverflow=on  OutDataTypeStr=Inherit: Same as input  ParamDataTypeStr=Inherit: Same as input
  Rad to Deg1 : Gain  Gain=180/pi  SaturateOnIntegerOverflow=on  OutDataTypeStr=Inherit: Same as input  ParamDataTypeStr=Inherit: Same as input
  Trigonometric Function : Trigonometry  Operator=atan2
  Trigonometric Function1 : Trigonometry  Operator=asin
  Alpha(deg) : Outport
  Beta(deg) : Outport  Port=2
  V : Outport  Port=3
  wires:
  Add/1 -> Dot Product/2, Dot Product/1, Demux/1
  Vb/1 -> Add/1
  Wind_b/1 -> Add/2
  Demux/2 -> Product/2
  Math Function/1 -> V/1, Product/1
  Product/1 -> Trigonometric Function1/1
  Demux/3 -> Trigonometric Function/1
  Demux/1 -> Trigonometric Function/2
  Dot Product/1 -> Math Function/1
  Trigonometric Function/1 -> Rad to Deg/1
  Rad to Deg/1 -> Alpha(deg)/1
  Trigonometric Function1/1 -> Rad to Deg1/1
  Rad to Deg1/1 -> Beta(deg)/1

== system gtm_design/GTM_T2/AuxiliaryVariables/VecNorm ==
  I : Inport
  Math Function2 : Math  Operator=sqrt  SignedPower=on  SaturateOnIntegerOverflow=on
  Product : Product  RndMeth=Zero
  Sum of Elements : Sum  Inputs=+
  O : Outport
  wires:
  Math Function2/1 -> O/1
  I/1 -> Product/1, Product/2
  Product/1 -> Sum of Elements/1
  Sum of Elements/1 -> Math Function2/1

== system gtm_design/GTM_T2/AuxiliaryVariables/WindShear and Xform ==
  Winds : Inport
  DCM : Inport  Port=2
  State : Inport  Port=3
  Add : Sum
  Add1 : Sum  Inputs=+-
  Bus Selector : BusSelector  OutputSignals=NorthWind,EastWind,VerticalWind  OutputAsBus=on
  Bus Selector1 : BusSelector  OutputSignals=turb_u_body,turb_v_body,turb_w_body  OutputAsBus=on
  Bus Selector11 : BusSelector  OutputSignals=altitude
  Bus to Vector : BusToVector
  Bus to Vector1 : BusToVector
  Constant : Constant  Value=WindShearOn
  Constant1 : Constant
  Constant2 : Constant  Value=runway_alt
  NED_Body : Product  Multiplication=Matrix(*)  RndMeth=Zero
  Scale : Product  Inputs=**
  Switch : Switch  Threshold=0.5
  WindShear : Subsystem
  BodyAxis Winds : Outport
  wires:
  WindShear/1(Out) -> Switch/1
  Switch/1 -> Scale/1
  Constant1/1 -> Switch/3
  Constant/1 -> Switch/2
  Add1/1 -> WindShear/1(In)
  Constant2/1 -> Add1/2
  Bus Selector11/1 -> Add1/1  "<altitude>"
  State/1 -> Bus Selector11/1
  Scale/1 -> Add/1  "SteadyWind"
  NED_Body/1 -> Scale/2
  Bus to Vector1/1 -> Add/2  "Turbulence"
  Add/1 -> BodyAxis Winds/1
  Bus Selector1/1 -> Bus to Vector1/1
  DCM/1 -> NED_Body/1
  Bus to Vector/1 -> NED_Body/2
  Bus Selector/1 -> Bus to Vector/1
  Winds/1 -> Bus Selector1/1, Bus Selector/1

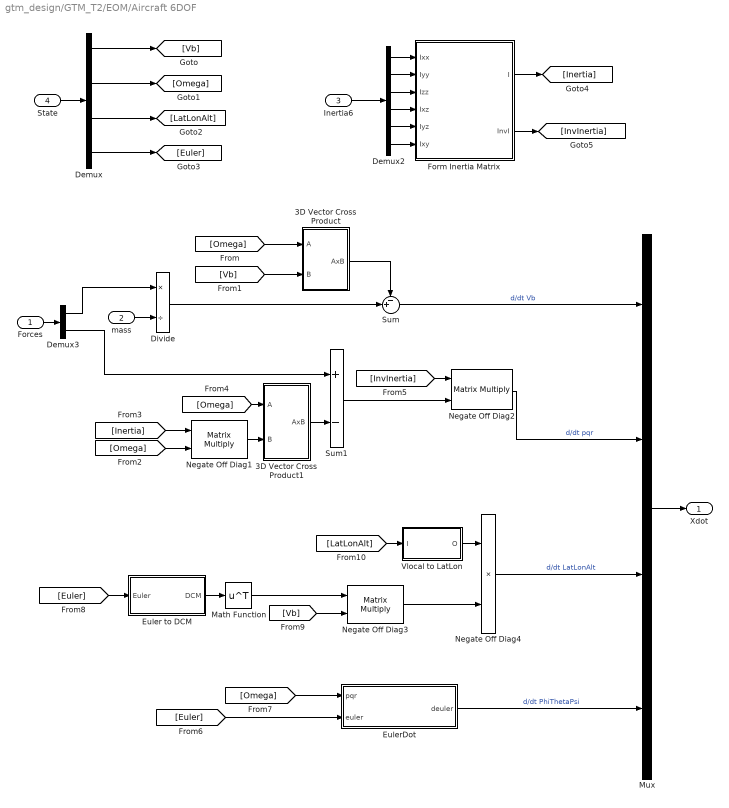
== system gtm_design/GTM_T2/EOM/Aircraft 6DOF ==
  Forces : Inport  PortDimensions=6
  mass : Inport  Port=2  PortDimensions=1
  Inertia6 : Inport  Port=3  PortDimensions=6
  State : Inport  Port=4  PortDimensions=12
  3D Vector Cross Product : Subsystem
  3D Vector Cross Product1 : Subsystem
  Demux : Demux  Outputs=[3 3 3 3]
  Demux2 : Demux  Outputs=6
  Demux3 : Demux  Outputs=[3 3]
  Divide : Product  Inputs=*/
  Euler to DCM : Subsystem
  EulerDot : MATLAB Function  TreatAsAtomicUnit=on
  Form Inertia Matrix : MATLAB Function  TreatAsAtomicUnit=on
  Math Function : Math  Operator=transpose  SignedPower=on  SaturateOnIntegerOverflow=on
  Mux : Mux
  Negate Off Diag1 : Product  Inputs=**  Multiplication=Matrix(*)
  Negate Off Diag2 : Product  Inputs=**  Multiplication=Matrix(*)
  Negate Off Diag3 : Product  Inputs=**  Multiplication=Matrix(*)
  Negate Off Diag4 : Product  Inputs=**
  Sum : Sum  Inputs=-+|  SaturateOnIntegerOverflow=on
  Sum1 : Sum  Inputs=+-  SaturateOnIntegerOverflow=on
  Vlocal to LatLon : Subsystem
  Xdot : Outport
  wires:
  Negate Off Diag3/1 -> Negate Off Diag4/2
  Demux2/6 -> Form Inertia Matrix/6(Ixy)
  Demux2/5 -> Form Inertia Matrix/5(Iyz)
  Form Inertia Matrix/1(I) -> [Inertia]
  Form Inertia Matrix/2(InvI) -> [InvInertia]
  Inertia6/1 -> Demux2/1
  Demux2/4 -> Form Inertia Matrix/4(Ixz)
  Demux2/3 -> Form Inertia Matrix/3(Izz)
  Demux2/2 -> Form Inertia Matrix/2(Iyy)
  Demux2/1 -> Form Inertia Matrix/1(Ixx)
  EulerDot/1(deuler) -> Mux/4  "d/dt PhiThetaPsi"
  Sum/1 -> Mux/1  "d/dt Vb"
  Forces/1 -> Demux3/1
  Demux3/1 -> Divide/1
  mass/1 -> Divide/2
  Demux3/2 -> Sum1/1
  [Omega] -> 3D Vector Cross Product/1(A)
  [Vb] -> 3D Vector Cross Product/2(B)
  [Omega] -> Negate Off Diag1/2
  [Inertia] -> Negate Off Diag1/1
  Negate Off Diag1/1 -> 3D Vector Cross Product1/2(B)
  [Omega] -> 3D Vector Cross Product1/1(A)
  3D Vector Cross Product1/1(AxB) -> Sum1/2
  Sum1/1 -> Negate Off Diag2/2
  [InvInertia] -> Negate Off Diag2/1
  Negate Off Diag2/1 -> Mux/2  "d/dt pqr"
  [Euler] -> EulerDot/2(euler)
  [Omega] -> EulerDot/1(pqr)
  [Euler] -> Euler to DCM/1("Euler ")
  Euler to DCM/1(DCM) -> Math Function/1
  [Vb] -> Negate Off Diag3/2
  [LatLonAlt] -> Vlocal to LatLon/1(I)
  Vlocal to LatLon/1(O) -> Negate Off Diag4/1
  Negate Off Diag4/1 -> Mux/3  "d/dt LatLonAlt"
  3D Vector Cross Product/1(AxB) -> Sum/1
  Divide/1 -> Sum/2
  State/1 -> Demux/1
  Demux/1 -> [Vb]
  Demux/2 -> [Omega]
  Demux/3 -> [LatLonAlt]
  Demux/4 -> [Euler]
  Math Function/1 -> Negate Off Diag3/1
  Mux/1 -> Xdot/1

== system gtm_design/GTM_T2/EOM/Anti Windup ==
  I : Inport
  Demux : Demux  Outputs=12
      settings: DisplayOption=none
  Mux : Mux  Inputs=12
  Subsystem1 : Subsystem
      mask Display: disp('no windup 180')
  Subsystem3 : Subsystem
      mask Display: disp('no windup 180')
  Subsystem4 : Subsystem
      mask Display: disp('no windup 360')
  O : Outport
  wires:
  Mux/1 -> O/1
  Demux/11 -> Subsystem1/1(I)  "theta"
  Demux/10 -> Subsystem3/1(I)  "phi"
  Subsystem4/1(O) -> Mux/12  "psi"
  Subsystem1/1(O) -> Mux/11  "theta"
  Subsystem3/1(O) -> Mux/10  "phi"
  I/1 -> Demux/1
  Demux/1 -> Mux/1  "ub"
  Demux/2 -> Mux/2  "vb"
  Demux/3 -> Mux/3  "wb"
  Demux/4 -> Mux/4  "pb"
  Demux/5 -> Mux/5  "qb"
  Demux/6 -> Mux/6  "rb"
  Demux/7 -> Mux/7  "latitude"
  Demux/8 -> Mux/8  "longitude"
  Demux/9 -> Mux/9  "altitude"
  Demux/12 -> Subsystem4/1(I)  "psi"

== system gtm_design/GTM_T2/EOM/State Labels ==
  I : Inport
  Bus Creator : BusCreator  Inputs=12
  Demux : Demux  Outputs=12
      settings: DisplayOption=none
  O : Outport
  wires:
  Demux/12 -> Bus Creator/12  "psi"
  Demux/9 -> Bus Creator/9  "altitude"
  Demux/8 -> Bus Creator/8  "longitude"
  Demux/7 -> Bus Creator/7  "latitude"
  Demux/6 -> Bus Creator/6  "rb"
  Demux/5 -> Bus Creator/5  "qb"
  Demux/4 -> Bus Creator/4  "pb"
  Demux/3 -> Bus Creator/3  "wb"
  Demux/2 -> Bus Creator/2  "vb"
  Demux/1 -> Bus Creator/1  "ub"
  I/1 -> Demux/1
  Demux/10 -> Bus Creator/10  "phi"
  Demux/11 -> Bus Creator/11  "theta"
  Bus Creator/1 -> O/1

== system gtm_design/GTM_T2/EOM/Xdot Labels ==
  I : Inport
  Bus Creator : BusCreator  Inputs=12
  Demux : Demux  Outputs=12
      settings: DisplayOption=none
  O : Outport
  wires:
  Bus Creator/1 -> O/1
  Demux/11 -> Bus Creator/11  "theta_dot"
  Demux/10 -> Bus Creator/10  "phi_dot"
  I/1 -> Demux/1
  Demux/1 -> Bus Creator/1  "ub_dot"
  Demux/2 -> Bus Creator/2  "vb_dot"
  Demux/3 -> Bus Creator/3  "wb_dot"
  Demux/4 -> Bus Creator/4  "pb_dot"
  Demux/5 -> Bus Creator/5  "qb_dot"
  Demux/6 -> Bus Creator/6  "rb_dot"
  Demux/7 -> Bus Creator/7  "latitude_dot"
  Demux/8 -> Bus Creator/8  "longitude_dot"
  Demux/9 -> Bus Creator/9  "altitude_dot"
  Demux/12 -> Bus Creator/12  "psi_dot"

== system gtm_design/GTM_T2/Engines/3D Vector Cross Product ==
  A : Inport
  B : Inport  Port=2
  Demux : Demux  Outputs=3
      settings: DisplayOption=none
  Demux1 : Demux  Outputs=3
      settings: DisplayOption=none
  Gain : Gain  Gain=-1  SaturateOnIntegerOverflow=on  OutDataTypeStr=Inherit: Same as input  ParamDataTypeStr=Inherit: Same as input
  Ground : Ground
  Mux : Mux  Inputs=9
  Product : Product  Multiplication=Matrix(*)  SaturateOnIntegerOverflow=on  OutDataTypeStr=Inherit: Same as first input
  Reshape : Reshape  OutputDimensionality=Customize  OutputDimensions=[3,3]
  AxB : Outport
  wires:
  A/1 -> Demux/1, Gain/1
  Product/1 -> AxB/1
  Ground/1 -> Mux/1, Mux/5, Mux/9
  Gain/1 -> Demux1/1
  Demux/3 -> Mux/2
  Demux1/2 -> Mux/3
  Demux1/3 -> Mux/4
  Demux/1 -> Mux/6
  Demux/2 -> Mux/7
  Demux1/1 -> Mux/8
  Mux/1 -> Reshape/1
  Reshape/1 -> Product/1
  B/1 -> Product/2

== system gtm_design/GTM_T2/Engines/CG torque ==
  AC : Inport
  Lthrust : Inport  Port=2
  Rthrust : Inport  Port=3
  3D Vector Cross Product : Subsystem
  3D Vector Cross Product1 : Subsystem
  Bus Selector30 : BusSelector  OutputSignals=LfEng,CG,RtEng
  Sum1 : Sum  InputSameDT=on  SaturateOnIntegerOverflow=on  OutDataTypeStr=Inherit: Same as first input
  Sum6 : Sum  Inputs=+-  InputSameDT=on  SaturateOnIntegerOverflow=on  OutDataTypeStr=Inherit: Same as first input
  Sum7 : Sum  Inputs=-+  InputSameDT=on  SaturateOnIntegerOverflow=on  OutDataTypeStr=Inherit: Same as first input
  Torques : Outport
  wires:
  AC/1 -> Bus Selector30/1
  Bus Selector30/2 -> Sum7/1, Sum6/2  "<CG>"
  Lthrust/1 -> 3D Vector Cross Product1/2(B)
  Rthrust/1 -> 3D Vector Cross Product/2(B)
  Sum7/1 -> 3D Vector Cross Product/1(A)
  Sum6/1 -> 3D Vector Cross Product1/1(A)
  3D Vector Cross Product1/1(AxB) -> Sum1/1
  3D Vector Cross Product/1(AxB) -> Sum1/2
  Sum1/1 -> Torques/1
  Bus Selector30/3 -> Sum7/2  "<RtEng>"
  Bus Selector30/1 -> Sum6/1  "<LfEng>"

== system gtm_design/GTM_T2/Engines/Left_Engine Jetcat P70 ==
  Throttle : Inport
  pratio : Inport  Port=2
  tratio : Inport  Port=3
  BypassDynamics : Inport  Port=4
  qbar : Inport  Port=5
  S : Inport  Port=6
  Display : Display
  Display1 : Display
  Fuel Pump Voltage : Lookup  InputValues=fuelflow_table  Table=fuelpump_table  LookUpMeth=Interpolation-Use End Values
  Product2 : Product  RndMeth=Zero
  RPMref_2_EGT : Polyval  Coefs=Coeff_EGT
  RPMref_2_FuelFlow : Polyval  Coefs=Coeff_fuelflow
  RPMref_2_Thrust : Polyval  Coefs=Coeff_thrust
  Saturation : Saturate  UpperLimit=inf  LowerLimit=0
  Simple Ram Drag Model : MATLAB Function  TreatAsAtomicUnit=on
  Sum : Sum  Inputs=-+|
  Switch : Switch  Criteria=u2 ~= 0
  Terminator : Terminator
  Throttle Lag1 : Subsystem
  Throttle2 : InportShadow
  Throttle_2_RPMref : Polyval  Coefs=Coeff_throttle
  To Workspace1 : ToWorkspace  VariableName=Throttle  SampleTime=-1
  UnScale_Ref_RPM : Gain  Gain=123000/100
  angular momentum : Gain  Gain=(pi*shaft_dia^4/32) * shaft_len * density * (2*pi/60)
  Thrust (lbf) : Outport
  RPM : Outport  Port=2
  h (slg-ft^2/s) : Outport  Port=3
  Fuel Pump Voltage (V) : Outport  Port=4
  EGT (deg C) : Outport  Port=5
  Fuel Flow (lbs/min) : Outport  Port=6
  wires:
  Saturation/1 -> Thrust (lbf)/1
  Sum/1 -> Saturation/1
  Product2/1 -> Display1/1, Sum/2
  Simple Ram Drag Model/1(ram_drag) -> Sum/1, Display/1
  S/1 -> Simple Ram Drag Model/2(S)
  qbar/1 -> Simple Ram Drag Model/1(qbar)
  Throttle2/1 -> Switch/1
  BypassDynamics/1 -> Switch/2
  Throttle Lag1/1(y) -> Switch/3  "Throttle_Lag"
  Switch/1 -> To Workspace1/1, Throttle_2_RPMref/1
  Throttle/1 -> Throttle Lag1/1(throttle)
  Throttle_2_RPMref/1 -> RPMref_2_Thrust/1, UnScale_Ref_RPM/1, RPMref_2_EGT/1, RPMref_2_FuelFlow/1
  angular momentum/1 -> h (slg-ft^2/s)/1
  UnScale_Ref_RPM/1 -> angular momentum/1, RPM/1
  tratio/1 -> Terminator/1
  RPMref_2_Thrust/1 -> Product2/1
  RPMref_2_FuelFlow/1 -> Fuel Flow (lbs/min)/1, Fuel Pump Voltage/1
  pratio/1 -> Product2/2
  Fuel Pump Voltage/1 -> Fuel Pump Voltage (V)/1
  RPMref_2_EGT/1 -> EGT (deg C)/1
